simulink model "sparrow_albatros_spec_withgpio"  (R2021a)
settings: Solver=VariableStepDiscrete  StartTime=0.0  StopTime=100  RelTol=1e-3
undefined symbols (not defined in the file): pfb_coeff_gen_calc
libraries: xbsIndex_r4 x5582, casper_library_misc x33, casper_library_delays x28, xps_library x10, simulink x8, xbsReplacements_r4 x2
(part 55 of 80)

== system sparrow_albatros_spec_withgpio/fft_wideband_real/fft_biplex_real_4x/biplex_core/fft_stage_7/butterfly_direct/bus_norm0 ==
  din : Inport
  bussify : Subsystem  AncestorBlock=casper_library_flow_control/bus_create  mask(bus_create){inputNum=4}
      mask prompts: inputNum "Number of inputs:"
      mask init:
      | bus_create_init(gcb,...
      |     'inputNum', inputNum);
  conv{1..4} (4 alike) : xbsIndex_r4/Convert  gui_display_data_type=Fixed-point  arith_type="Signed  (2's comp)"  n_bits=27  bin_pt=18  float_type=Single  exp_bits=8  fraction_bits=24  quantization=Truncate  overflow=Wrap  en=off  latency=0  pipeline=on  dbl_ovrd=off  block_type=convert
  debus : Subsystem  AncestorBlock=casper_library_flow_control/bus_expand  mask(bus_expand){mode=divisions of arbitrary size, outputNum=2, outputWidth=[26 26 26 26], outputBinaryPt=[17 17 17 17], outputArithmeticType=[1 1 1 1], show_format=on, outputToWorkspace=off, variablePrefix=, outputToModelAsWell=on}
      mask prompts: outputNum "Number of outputs:"; outputWidth "Output width:"; outputBinaryPt "Output binary point position:"; outputArithmeticType "Output arithmetic type (ufix=0, fix=1, bool=2):"; show_format "Print format string?"; outputToWorkspace "Output to workspace?"; variablePrefix "Variable name prefix:"; outputToModelAsWell "Output to model as well?"
      mask help:
      | Expands a 'bus' made using a bus_create or Xilinx
      | concat block.
      | The input will be divided into the specified number
      | of outputs with the specified arithmetic types.
      | Divisions are made from most significant bit.
      mask init: same as sparrow_albatros_spec_withgpio/bus_expand
      settings: AttributesFormatString=4 outputs: f26.17,f26.17,f26.17,f26.17,
      mask TypeOptions mode: divisions of equal size | divisions of arbitrary size
      mask Callback mode: %bus_expand_callback();
      mask Callback outputWidth: %bus_expand_callback();
      mask Callback outputToWorkspace: %bus_expand_callback();
  dout : Outport
  wires:
  din/1 -> debus/1(bus_in)
  debus/1(msb_out4) -> conv1/1
  debus/2(out3) -> conv2/1
  debus/3(out2) -> conv3/1
  debus/4(lsb_out1) -> conv4/1
  conv1/1 -> bussify/1(in1)
  conv2/1 -> bussify/2(in2)
  conv3/1 -> bussify/3(in3)
  conv4/1 -> bussify/4(in4)
  bussify/1(bus_out) -> dout/1

== system sparrow_albatros_spec_withgpio/fft_wideband_real/fft_biplex_real_4x/biplex_core/fft_stage_7/butterfly_direct/bus_norm1 ==
  din : Inport
  bussify : Subsystem  AncestorBlock=casper_library_flow_control/bus_create  mask(bus_create){inputNum=4}
      mask prompts: inputNum "Number of inputs:"
      mask init:
      | bus_create_init(gcb,...
      |     'inputNum', inputNum);
  conv{1..4} (4 alike) : xbsIndex_r4/Convert  gui_display_data_type=Fixed-point  arith_type="Signed  (2's comp)"  n_bits=27  bin_pt=18  float_type=Single  exp_bits=8  fraction_bits=24  quantization=Truncate  overflow=Wrap  en=off  latency=0  pipeline=on  dbl_ovrd=off  block_type=convert
  debus : Subsystem  AncestorBlock=casper_library_flow_control/bus_expand  mask(bus_expand){mode=divisions of arbitrary size, outputNum=2, outputWidth=[26 26 26 26], outputBinaryPt=[18 18 18 18], outputArithmeticType=[1 1 1 1], show_format=on, outputToWorkspace=off, variablePrefix=, outputToModelAsWell=on}
      mask prompts: outputNum "Number of outputs:"; outputWidth "Output width:"; outputBinaryPt "Output binary point position:"; outputArithmeticType "Output arithmetic type (ufix=0, fix=1, bool=2):"; show_format "Print format string?"; outputToWorkspace "Output to workspace?"; variablePrefix "Variable name prefix:"; outputToModelAsWell "Output to model as well?"
      mask help:
      | Expands a 'bus' made using a bus_create or Xilinx
      | concat block.
      | The input will be divided into the specified number
      | of outputs with the specified arithmetic types.
      | Divisions are made from most significant bit.
      mask init: same as sparrow_albatros_spec_withgpio/bus_expand
      settings: AttributesFormatString=4 outputs: f26.18,f26.18,f26.18,f26.18,
      mask TypeOptions mode: divisions of equal size | divisions of arbitrary size
      mask Callback mode: %bus_expand_callback();
      mask Callback outputWidth: %bus_expand_callback();
      mask Callback outputToWorkspace: %bus_expand_callback();
  dout : Outport
  wires:
  din/1 -> debus/1(bus_in)
  debus/1(msb_out4) -> conv1/1
  debus/2(out3) -> conv2/1
  debus/3(out2) -> conv3/1
  debus/4(lsb_out1) -> conv4/1
  conv1/1 -> bussify/1(in1)
  conv2/1 -> bussify/2(in2)
  conv3/1 -> bussify/3(in3)
  conv4/1 -> bussify/4(in4)
  bussify/1(bus_out) -> dout/1

== system sparrow_albatros_spec_withgpio/fft_wideband_real/fft_biplex_real_4x/biplex_core/fft_stage_7/butterfly_direct/bus_relational ==
  a : Inport
  b : Inport  Port=2
  a_debus : Subsystem  AncestorBlock=casper_library_flow_control/bus_expand  mask(bus_expand){mode=divisions of arbitrary size, outputNum=2, outputWidth=[4], outputBinaryPt=[0], outputArithmeticType=[0], show_format=on, outputToWorkspace=off, variablePrefix=, outputToModelAsWell=on}
      mask prompts: outputNum "Number of outputs:"; outputWidth "Output width:"; outputBinaryPt "Output binary point position:"; outputArithmeticType "Output arithmetic type (ufix=0, fix=1, bool=2):"; show_format "Print format string?"; outputToWorkspace "Output to workspace?"; variablePrefix "Variable name prefix:"; outputToModelAsWell "Output to model as well?"
      mask help:
      | Expands a 'bus' made using a bus_create or Xilinx
      | concat block.
      | The input will be divided into the specified number
      | of outputs with the specified arithmetic types.
      | Divisions are made from most significant bit.
      mask init: same as sparrow_albatros_spec_withgpio/bus_expand
      settings: AttributesFormatString=1 outputs: uf4.0,
      mask TypeOptions mode: divisions of equal size | divisions of arbitrary size
      mask Callback mode: %bus_expand_callback();
      mask Callback outputWidth: %bus_expand_callback();
      mask Callback outputToWorkspace: %bus_expand_callback();
  b_debus : Subsystem  AncestorBlock=casper_library_flow_control/bus_expand  mask(bus_expand){mode=divisions of arbitrary size, outputNum=2, outputWidth=[4], outputBinaryPt=[0], outputArithmeticType=[0], show_format=on, outputToWorkspace=off, variablePrefix=, outputToModelAsWell=on}
      mask prompts: outputNum "Number of outputs:"; outputWidth "Output width:"; outputBinaryPt "Output binary point position:"; outputArithmeticType "Output arithmetic type (ufix=0, fix=1, bool=2):"; show_format "Print format string?"; outputToWorkspace "Output to workspace?"; variablePrefix "Variable name prefix:"; outputToModelAsWell "Output to model as well?"
      mask help:
      | Expands a 'bus' made using a bus_create or Xilinx
      | concat block.
      | The input will be divided into the specified number
      | of outputs with the specified arithmetic types.
      | Divisions are made from most significant bit.
      mask init: same as sparrow_albatros_spec_withgpio/bus_expand
      settings: AttributesFormatString=1 outputs: uf4.0,
      mask TypeOptions mode: divisions of equal size | divisions of arbitrary size
      mask Callback mode: %bus_expand_callback();
      mask Callback outputWidth: %bus_expand_callback();
      mask Callback outputToWorkspace: %bus_expand_callback();
  bussify : Subsystem  AncestorBlock=casper_library_flow_control/bus_create  mask(bus_create){inputNum=1}
      mask prompts: inputNum "Number of inputs:"
      mask init:
      | bus_create_init(gcb,...
      |     'inputNum', inputNum);
  relational1 : xbsIndex_r4/Relational  mode=a!=b  op_type=Bool  en=off  latency=1  dbl_ovrd=off  block_type=relational
  a!=b : Outport
  wires:
  a/1 -> a_debus/1(bus_in)
  b/1 -> b_debus/1(bus_in)
  a_debus/1(msb_lsb_out1) -> relational1/1
  b_debus/1(msb_lsb_out1) -> relational1/2
  relational1/1 -> bussify/1(in1)
  bussify/1(bus_out) -> a!=b/1

== system sparrow_albatros_spec_withgpio/fft_wideband_real/fft_biplex_real_4x/biplex_core/fft_stage_7/butterfly_direct/bus_scale ==
  din : Inport
  bussify : Subsystem  AncestorBlock=casper_library_flow_control/bus_create  mask(bus_create){inputNum=4}
      mask prompts: inputNum "Number of inputs:"
      mask init:
      | bus_create_init(gcb,...
      |     'inputNum', inputNum);
  debus : Subsystem  AncestorBlock=casper_library_flow_control/bus_expand  mask(bus_expand){mode=divisions of arbitrary size, outputNum=2, outputWidth=[26 26 26 26], outputBinaryPt=[17 17 17 17], outputArithmeticType=[1 1 1 1], show_format=on, outputToWorkspace=off, variablePrefix=, outputToModelAsWell=on}
      mask prompts: outputNum "Number of outputs:"; outputWidth "Output width:"; outputBinaryPt "Output binary point position:"; outputArithmeticType "Output arithmetic type (ufix=0, fix=1, bool=2):"; show_format "Print format string?"; outputToWorkspace "Output to workspace?"; variablePrefix "Variable name prefix:"; outputToModelAsWell "Output to model as well?"
      mask help:
      | Expands a 'bus' made using a bus_create or Xilinx
      | concat block.
      | The input will be divided into the specified number
      | of outputs with the specified arithmetic types.
      | Divisions are made from most significant bit.
      mask init: same as sparrow_albatros_spec_withgpio/bus_expand
      settings: AttributesFormatString=4 outputs: f26.17,f26.17,f26.17,f26.17,
      mask TypeOptions mode: divisions of equal size | divisions of arbitrary size
      mask Callback mode: %bus_expand_callback();
      mask Callback outputWidth: %bus_expand_callback();
      mask Callback outputToWorkspace: %bus_expand_callback();
  scale{1..4} (4 alike) : xbsIndex_r4/Scale  scale_factor=-1  dbl_ovrd=off  block_type=scale
  dout : Outport
  wires:
  din/1 -> debus/1(bus_in)
  debus/1(msb_out4) -> scale1/1
  debus/2(out3) -> scale2/1
  debus/3(out2) -> scale3/1
  debus/4(lsb_out1) -> scale4/1
  scale1/1 -> bussify/1(in1)
  scale2/1 -> bussify/2(in2)
  scale3/1 -> bussify/3(in3)
  scale4/1 -> bussify/4(in4)
  bussify/1(bus_out) -> dout/1

== system sparrow_albatros_spec_withgpio/fft_wideband_real/fft_biplex_real_4x/biplex_core/fft_stage_7/butterfly_direct/bus_sub ==
  a : Inport
  b : Inport  Port=2
  a_debus : Subsystem  AncestorBlock=casper_library_flow_control/bus_expand  mask(bus_expand){mode=divisions of arbitrary size, outputNum=2, outputWidth=[24  24], outputBinaryPt=[17  17], outputArithmeticType=[1  1], show_format=on, outputToWorkspace=off, variablePrefix=, outputToModelAsWell=on}
      mask prompts: outputNum "Number of outputs:"; outputWidth "Output width:"; outputBinaryPt "Output binary point position:"; outputArithmeticType "Output arithmetic type (ufix=0, fix=1, bool=2):"; show_format "Print format string?"; outputToWorkspace "Output to workspace?"; variablePrefix "Variable name prefix:"; outputToModelAsWell "Output to model as well?"
      mask help:
      | Expands a 'bus' made using a bus_create or Xilinx
      | concat block.
      | The input will be divided into the specified number
      | of outputs with the specified arithmetic types.
      | Divisions are made from most significant bit.
      mask init: same as sparrow_albatros_spec_withgpio/bus_expand
      settings: AttributesFormatString=2 outputs: f24.17,f24.17,
      mask TypeOptions mode: divisions of equal size | divisions of arbitrary size
      mask Callback mode: %bus_expand_callback();
      mask Callback outputWidth: %bus_expand_callback();
      mask Callback outputToWorkspace: %bus_expand_callback();
  addsub1 : xbsIndex_r4/AddSub  mode=Subtraction  use_carryin=off  use_carryout=off  en=off  latency=1  precision=User Defined  arith_type="Signed  (2's comp)"  n_bits=26  bin_pt=17  quantization=Truncate  overflow=Wrap  use_behavioral_HDL=on  hw_selection=Fabric  pipelined=on  dbl_ovrd=off  block_type=addsub
  addsub2 : xbsIndex_r4/AddSub  mode=Subtraction  use_carryin=off  use_carryout=off  en=off  latency=1  precision=User Defined  arith_type="Signed  (2's comp)"  n_bits=26  bin_pt=17  quantization=Truncate  overflow=Wrap  use_behavioral_HDL=on  hw_selection=Fabric  pipelined=on  dbl_ovrd=off  block_type=addsub
  b_debus : Subsystem  AncestorBlock=casper_library_flow_control/bus_expand  mask(bus_expand){mode=divisions of arbitrary size, outputNum=2, outputWidth=[25  25], outputBinaryPt=[17  17], outputArithmeticType=[1  1], show_format=on, outputToWorkspace=off, variablePrefix=, outputToModelAsWell=on}
      mask prompts: outputNum "Number of outputs:"; outputWidth "Output width:"; outputBinaryPt "Output binary point position:"; outputArithmeticType "Output arithmetic type (ufix=0, fix=1, bool=2):"; show_format "Print format string?"; outputToWorkspace "Output to workspace?"; variablePrefix "Variable name prefix:"; outputToModelAsWell "Output to model as well?"
      mask help:
      | Expands a 'bus' made using a bus_create or Xilinx
      | concat block.
      | The input will be divided into the specified number
      | of outputs with the specified arithmetic types.
      | Divisions are made from most significant bit.
      mask init: same as sparrow_albatros_spec_withgpio/bus_expand
      settings: AttributesFormatString=2 outputs: f25.17,f25.17,
      mask TypeOptions mode: divisions of equal size | divisions of arbitrary size
      mask Callback mode: %bus_expand_callback();
      mask Callback outputWidth: %bus_expand_callback();
      mask Callback outputToWorkspace: %bus_expand_callback();
  op_bussify : Subsystem  AncestorBlock=casper_library_flow_control/bus_create  mask(bus_create){inputNum=2}
      mask prompts: inputNum "Number of inputs:"
      mask init:
      | bus_create_init(gcb,...
      |     'inputNum', inputNum);
  dout : Outport
  wires:
  a/1 -> a_debus/1(bus_in)
  b/1 -> b_debus/1(bus_in)
  a_debus/1(msb_out2) -> addsub1/1
  b_debus/1(msb_out2) -> addsub1/2
  a_debus/2(lsb_out1) -> addsub2/1
  b_debus/2(lsb_out1) -> addsub2/2
  addsub1/1 -> op_bussify/1(in1)
  addsub2/1 -> op_bussify/2(in2)
  op_bussify/1(bus_out) -> dout/1

== system sparrow_albatros_spec_withgpio/fft_wideband_real/fft_biplex_real_4x/biplex_core/fft_stage_7/butterfly_direct/munge ==
  din : Inport
  join : Subsystem  AncestorBlock=casper_library_flow_control/bus_create  mask(bus_create){inputNum=2}
      mask prompts: inputNum "Number of inputs:"
      mask init:
      | bus_create_init(gcb,...
      |     'inputNum', inputNum);
  reinterpret : xbsIndex_r4/Reinterpret  force_arith_type=on  arith_type=Unsigned  force_bin_pt=on  bin_pt=0  block_type=reinterpret
  reinterpret_out : xbsIndex_r4/Reinterpret  force_arith_type=on  arith_type=Unsigned  force_bin_pt=on  bin_pt=0  block_type=reinterpret
  split : Subsystem  AncestorBlock=casper_library_flow_control/bus_expand  mask(bus_expand){mode=divisions of arbitrary size, outputNum=2, outputWidth=[2 2], outputBinaryPt=[0 0], outputArithmeticType=[0 0], show_format=off, outputToWorkspace=off, variablePrefix=out, outputToModelAsWell=on}
      mask prompts: outputNum "Number of outputs:"; outputWidth "Output width:"; outputBinaryPt "Output binary point position:"; outputArithmeticType "Output arithmetic type (ufix=0, fix=1, bool=2):"; show_format "Print format string?"; outputToWorkspace "Output to workspace?"; variablePrefix "Variable name prefix:"; outputToModelAsWell "Output to model as well?"
      mask help:
      | Expands a 'bus' made using a bus_create or Xilinx
      | concat block.
      | The input will be divided into the specified number
      | of outputs with the specified arithmetic types.
      | Divisions are made from most significant bit.
      mask init: same as sparrow_albatros_spec_withgpio/bus_expand
      settings: AttributesFormatString=2 outputs
      mask TypeOptions mode: divisions of equal size | divisions of arbitrary size
      mask Callback mode: %bus_expand_callback();
      mask Callback outputWidth: %bus_expand_callback();
      mask Callback outputToWorkspace: %bus_expand_callback();
  dout : Outport
  wires:
  reinterpret_out/1 -> dout/1
  din/1 -> reinterpret/1
  reinterpret/1 -> split/1(bus_in)
  join/1(bus_out) -> reinterpret_out/1
  split/1(msb_out2) -> join/1(in1)
  split/2(lsb_out1) -> join/2(in2)

== system sparrow_albatros_spec_withgpio/fft_wideband_real/fft_biplex_real_4x/biplex_core/fft_stage_7/butterfly_direct/mux ==
  sel : Inport
  d0 : Inport  Port=2
  d1 : Inport  Port=3
  d_bussify : Subsystem  AncestorBlock=casper_library_flow_control/bus_create  mask(bus_create){inputNum=4}
      mask prompts: inputNum "Number of inputs:"
      mask init:
      | bus_create_init(gcb,...
      |     'inputNum', inputNum);
  expand0 : Subsystem  AncestorBlock=casper_library_flow_control/bus_expand  mask(bus_expand){mode=divisions of arbitrary size, outputNum=2, outputWidth=[27 27 27 27], outputBinaryPt=[0  0  0  0], outputArithmeticType=[0  0  0  0], show_format=on, outputToWorkspace=off, variablePrefix=, outputToModelAsWell=on}
      mask prompts: outputNum "Number of outputs:"; outputWidth "Output width:"; outputBinaryPt "Output binary point position:"; outputArithmeticType "Output arithmetic type (ufix=0, fix=1, bool=2):"; show_format "Print format string?"; outputToWorkspace "Output to workspace?"; variablePrefix "Variable name prefix:"; outputToModelAsWell "Output to model as well?"
      mask help:
      | Expands a 'bus' made using a bus_create or Xilinx
      | concat block.
      | The input will be divided into the specified number
      | of outputs with the specified arithmetic types.
      | Divisions are made from most significant bit.
      mask init: same as sparrow_albatros_spec_withgpio/bus_expand
      settings: AttributesFormatString=4 outputs: uf27.0,uf27.0,uf27.0,uf27.0,
      mask TypeOptions mode: divisions of equal size | divisions of arbitrary size
      mask Callback mode: %bus_expand_callback();
      mask Callback outputWidth: %bus_expand_callback();
      mask Callback outputToWorkspace: %bus_expand_callback();
  expand1 : Subsystem  AncestorBlock=casper_library_flow_control/bus_expand  mask(bus_expand){mode=divisions of arbitrary size, outputNum=2, outputWidth=[27 27 27 27], outputBinaryPt=[0  0  0  0], outputArithmeticType=[0  0  0  0], show_format=on, outputToWorkspace=off, variablePrefix=, outputToModelAsWell=on}
      mask prompts: outputNum "Number of outputs:"; outputWidth "Output width:"; outputBinaryPt "Output binary point position:"; outputArithmeticType "Output arithmetic type (ufix=0, fix=1, bool=2):"; show_format "Print format string?"; outputToWorkspace "Output to workspace?"; variablePrefix "Variable name prefix:"; outputToModelAsWell "Output to model as well?"
      mask help:
      | Expands a 'bus' made using a bus_create or Xilinx
      | concat block.
      | The input will be divided into the specified number
      | of outputs with the specified arithmetic types.
      | Divisions are made from most significant bit.
      mask init: same as sparrow_albatros_spec_withgpio/bus_expand
      settings: AttributesFormatString=4 outputs: uf27.0,uf27.0,uf27.0,uf27.0,
      mask TypeOptions mode: divisions of equal size | divisions of arbitrary size
      mask Callback mode: %bus_expand_callback();
      mask Callback outputWidth: %bus_expand_callback();
      mask Callback outputToWorkspace: %bus_expand_callback();
  mux{0..3} (4 alike) : xbsIndex_r4/Mux  inputs=2  en=off  latency=1  precision=Full  arith_type=Unsigned  n_bits=16  bin_pt=14  quantization=Truncate  overflow=Wrap  dbl_ovrd=off  block_type=mux
  sel_expand : Subsystem  AncestorBlock=casper_library_flow_control/bus_expand  mask(bus_expand){mode=divisions of equal size, outputNum=4, outputWidth=1, outputBinaryPt=0, outputArithmeticType=0, show_format=on, outputToWorkspace=off, variablePrefix=, outputToModelAsWell=on}
      mask prompts: outputNum "Number of outputs:"; outputWidth "Output width:"; outputBinaryPt "Output binary point position:"; outputArithmeticType "Output arithmetic type (ufix=0, fix=1, bool=2):"; show_format "Print format string?"; outputToWorkspace "Output to workspace?"; variablePrefix "Variable name prefix:"; outputToModelAsWell "Output to model as well?"
      mask help:
      | Expands a 'bus' made using a bus_create or Xilinx
      | concat block.
      | The input will be divided into the specified number
      | of outputs with the specified arithmetic types.
      | Divisions are made from most significant bit.
      mask init: same as sparrow_albatros_spec_withgpio/bus_expand
      settings: AttributesFormatString=4 outputs: uf1.0,uf1.0,uf1.0,uf1.0,
      mask TypeOptions mode: divisions of equal size | divisions of arbitrary size
      mask Callback mode: %bus_expand_callback();
      mask Callback outputWidth: %bus_expand_callback();
      mask Callback outputToWorkspace: %bus_expand_callback();
  out : Outport
  wires:
  sel/1 -> sel_expand/1(bus_in)
  d0/1 -> expand0/1(bus_in)
  d1/1 -> expand1/1(bus_in)
  sel_expand/1(msb_out4) -> mux0/1
  expand0/1(msb_out4) -> mux0/2
  expand1/1(msb_out4) -> mux0/3
  sel_expand/2(out3) -> mux1/1
  expand0/2(out3) -> mux1/2
  expand1/2(out3) -> mux1/3
  sel_expand/3(out2) -> mux2/1
  expand0/3(out2) -> mux2/2
  expand1/3(out2) -> mux2/3
  sel_expand/4(lsb_out1) -> mux3/1
  expand0/4(lsb_out1) -> mux3/2
  expand1/4(lsb_out1) -> mux3/3
  mux0/1 -> d_bussify/1(in1)
  mux1/1 -> d_bussify/2(in2)
  mux2/1 -> d_bussify/3(in3)
  mux3/1 -> d_bussify/4(in4)
  d_bussify/1(bus_out) -> out/1

== system sparrow_albatros_spec_withgpio/fft_wideband_real/fft_biplex_real_4x/biplex_core/fft_stage_7/butterfly_direct/shift_replicate ==
  in : Inport
  bussify : Subsystem  AncestorBlock=casper_library_flow_control/bus_create  mask(bus_create){inputNum=4}
      mask prompts: inputNum "Number of inputs:"
      mask init:
      | bus_create_init(gcb,...
      |     'inputNum', inputNum);
  din0_{0..3} (4 alike) : xbsIndex_r4/Delay  rst=off  infoeditControl=Selection of Reset will increase slice count due to use of real FFs and instead of SRLs  en=off  latency=1  reg_retiming=off  dbl_ovrd=off  block_type=delay
  out : Outport
  wires:
  in/1 -> din0_0/1, din0_1/1, din0_2/1, din0_3/1
  din0_0/1 -> bussify/1(in1)
  din0_1/1 -> bussify/2(in2)
  din0_2/1 -> bussify/3(in3)
  din0_3/1 -> bussify/4(in4)
  bussify/1(bus_out) -> out/1

== system sparrow_albatros_spec_withgpio/fft_wideband_real/fft_biplex_real_4x/biplex_core/fft_stage_7/butterfly_direct/twiddle ==
  ai : Inport
  bi : Inport  Port=2
  sync_in : Inport  Port=3
  bus_convert : Subsystem  AncestorBlock=casper_library_bus/bus_convert  mask(bus_convert){n_bits_in=repmat(input_bit_width+coeff_bit_width+1, 1, n_inputs), bin_pt_in=(bin_pt_in+coeff_bit_width-1), cmplx=on, n_bits_out=input_bit_width+1, bin_pt_out=bin_pt_in, quantization=2, overflow=1, csp_latency=conv_latency, of=off, misc=on}
      mask prompts: n_bits_in "input bit widths"; bin_pt_in "input binary points"; cmplx "input complex"; n_bits_out "output bit widths"; bin_pt_out "output binary points"; quantization "quantization strategy (Truncate=0, Round  (unbiased: +/- Inf)=1, Round (unbiased: Even Values)=2)"; overflow "overflow strategy (Wrap=0, Saturate=1, Flag as error=2)"; csp_latency "latency"; of "overflow indication"; misc "misc support"
      mask help: Convert components of busses
      mask init: same as sparrow_albatros_spec_withgpio/tvg/bus_convert
  bus_create : Subsystem  AncestorBlock=casper_library_flow_control/bus_create  mask(bus_create){inputNum=3}
      mask prompts: inputNum "Number of inputs:"
      mask init:
      | bus_create_init(gcb,...
      |     'inputNum', inputNum);
  bus_expand : Subsystem  AncestorBlock=casper_library_flow_control/bus_expand  mask(bus_expand){mode=divisions of arbitrary size, outputNum=2, outputWidth=[n_inputs*input_bit_width*2, 1+(n_inputs*input_bit_width*2)], outputBinaryPt=[0 0], outputArithmeticType=[0 0], show_format=off, outputToWorkspace=off, variablePrefix=out, outputToModelAsWell=on}
      mask prompts: outputNum "Number of outputs:"; outputWidth "Output width:"; outputBinaryPt "Output binary point position:"; outputArithmeticType "Output arithmetic type (ufix=0, fix=1, bool=2):"; show_format "Print format string?"; outputToWorkspace "Output to workspace?"; variablePrefix "Variable name prefix:"; outputToModelAsWell "Output to model as well?"
      mask help:
      | Expands a 'bus' made using a bus_create or Xilinx
      | concat block.
      | The input will be divided into the specified number
      | of outputs with the specified arithmetic types.
      | Divisions are made from most significant bit.
      mask init: same as sparrow_albatros_spec_withgpio/bus_expand
      settings: AttributesFormatString=2 outputs
      mask TypeOptions mode: divisions of equal size | divisions of arbitrary size
      mask Callback mode: %bus_expand_callback();
      mask Callback outputWidth: %bus_expand_callback();
      mask Callback outputToWorkspace: %bus_expand_callback();
  bus_expand1 : Subsystem  AncestorBlock=casper_library_flow_control/bus_expand  mask(bus_expand){mode=divisions of arbitrary size, outputNum=2, outputWidth=[1 48], outputBinaryPt=[0 0], outputArithmeticType=[2 0], show_format=off, outputToWorkspace=off, variablePrefix=out, outputToModelAsWell=on}
      mask prompts: outputNum "Number of outputs:"; outputWidth "Output width:"; outputBinaryPt "Output binary point position:"; outputArithmeticType "Output arithmetic type (ufix=0, fix=1, bool=2):"; show_format "Print format string?"; outputToWorkspace "Output to workspace?"; variablePrefix "Variable name prefix:"; outputToModelAsWell "Output to model as well?"
      mask help:
      | Expands a 'bus' made using a bus_create or Xilinx
      | concat block.
      | The input will be divided into the specified number
      | of outputs with the specified arithmetic types.
      | Divisions are made from most significant bit.
      mask init: same as sparrow_albatros_spec_withgpio/bus_expand
      settings: AttributesFormatString=2 outputs
      mask TypeOptions mode: divisions of equal size | divisions of arbitrary size
      mask Callback mode: %bus_expand_callback();
      mask Callback outputWidth: %bus_expand_callback();
      mask Callback outputToWorkspace: %bus_expand_callback();
  bus_mult : Subsystem  AncestorBlock=casper_library_bus/bus_mult  mask(bus_mult){n_bits_a=coeff_bit_width, bin_pt_a=coeff_bit_width-1, type_a=1, cmplx_a=on, n_bits_b=24, bin_pt_b=bin_pt_in, type_b=1, cmplx_b=on, misc=on, floating_point=off, float_type=single, input_vec_a=1, input_vec_b=1, frac_width=24, exp_width=8, n_bits_out=input_bit_width+coeff_bit_width+1, bin_pt_out=(bin_pt_in+coeff_bit_width-1), type_out=1, quantization=0, overflow=0, mult_latency=mult_latency, add_latency=add_latency, conv_latency=0, max_fanout=max_fanout, fan_latency=0, multiplier_implementation=behavioral HDL, pipeline_cmult_en=off, pipeline_latency=0}
      mask prompts: n_bits_a "a input bit widths"; bin_pt_a "a input binary points"; type_a "a input type (Unsigned=0, Signed=1)"; cmplx_a "a input complex"; n_bits_b "b input bit widths"; bin_pt_b "b input binary points"; type_b "b input type (Unsigned=0, Signed=1)"; cmplx_b "b input complex"; misc "misc support"; floating_point "floating point"; float_type "float type"; input_vec_a "a input vector in bus"; input_vec_b "b input vector in bus"; frac_width "fraction width"; exp_width "exponent width"; n_bits_out "output bit widths"; bin_pt_out "output binary points"; type_out "output type (Unsigned=0, Signed=1)"; quantization "quantization strategy (Truncate=0, Round  (unbiased: +/- Inf)=1, , Round  (unbiased: Even Values)=2)"; overflow "overflow strategy (Wrap=0, Saturate=1, Flag as error=2)"; mult_latency "multiplier latency"; add_latency "adder latency"; conv_latency "convert latency"; max_fanout "limit fanout to ?"; fan_latency "fanout register latency"; multiplier_implementation "multiplier implementation"; pipeline_cmult_en "pipeline complex mult"; pipeline_latency "pipeline latency"
      mask help: Multiply components of two busses
      mask init: same as sparrow_albatros_spec_withgpio/fft_wideband_real/fft_direct/butterfly0_0/twiddle/bus_mult
      mask Callback floating_point:
      | onoff = get_param(gcb, 'floating_point');
      | if strcmp(onoff,'on')
      |     enable_fixpt = 'off';
      |     set_param_state(gcb, 'float_type', 'on')
      | 
      |     set_param_state(gcb, 'input_vec_a', 'on')
      |     set_param_state(gcb, 'input_vec_b', 'on')
      | 
      |     f_type = get_param(gcb, 'float_type');
      |     if strcmp(f_type,'custom')
      |         set_param_state(gcb, 'exp_width', 'on')
      |         set_param_state(gcb, 'frac_width', 'on')
      |     else
      |         set_param_state(gcb, 'exp_width', 'off')
      |         set_param_state(gcb, 'frac_width', 'off')
      |     end
      | 
      | else
      |     enable_fixpt = 'on';
      |     set_param_state(gcb, 'float_type', 'off')
      |     set_param_state(gcb, 'exp_width', 'off')
      |     set_param_state(gcb, 'frac_width', 'off')
      |     set_param_state(gcb, 'input_vec_a', 'off')
      |     set_param_state(gcb, 'input_vec_b', 'off')
      | end
      | 
      | set_param_state(gcb, 'n_bits_a', enable_fixpt)
      | set_param_state(gcb, 'bin_pt_a', enable_fixpt)
      | set_param_state(gcb, 'type_a', enable_fixpt)
      | set_param_state(gcb, 'n_bits_b', enable_fixpt)
      | set_param_state(gcb, 'bin_pt_b', enable_fixpt)
      | set_param_state(gcb, 'type_b', enable_fixpt)
      | 
      | set_param_state(gcb, 'n_bits_out', enable_fixpt)
      | set_param_state(gcb, 'bin_pt_out', enable_fixpt)
      | set_param_state(gcb, 'type_out', enable_fixpt)
      | set_param_state(gcb, 'quantization', enable_fixpt)
      | set_param_state(gcb, 'overflow', enable_fixpt)
      mask TypeOptions float_type: single | custom
      mask Callback float_type:
      | f_type = get_param(gcb, 'float_type');
      | if strcmp(f_type,'custom')
      |     set_param_state(gcb, 'exp_width', 'on')
      |     set_param_state(gcb, 'frac_width', 'on')
      | else
      |     set_param_state(gcb, 'exp_width', 'off')
      |     set_param_state(gcb, 'frac_width', 'off')
      | end
      mask TypeOptions multiplier_implementation: behavioral HDL | standard core | embedded multiplier core
      mask Callback pipeline_cmult_en:
      | pipeline_en = get_param(gcb, 'pipeline_cmult_en');
      | if strcmp(pipeline_en,'on')
      | 
      |     set_param_state(gcb, 'pipeline_latency', 'on')
      | else
      |     set_param_state(gcb, 'pipeline_latency', 'off')
      | end
  coeff_gen : Subsystem  AncestorBlock=casper_library_ffts_twiddle_coeff_gen/coeff_gen  mask(coeff_gen){FFTSize=FFTSize, Coeffs=[0 1 2 3 4 5 6 7 8 9 10 11 12 13 14 15 16 17 18 19 20 21 22 23 24 25 26 27 28 29 30 31 32 33 34 35 36 37 38 39 40 41 42 43 44 45 46 47 48 49 50 51 52 53 54 55 56 57 58 59 60 61 62 63], coeff_bit_width=coeff_bit_width, StepPeriod=StepPeriod, async=off, misc=on, floating_point=off, float_type=single, exp_width=8, frac_width=24, bram_latency=bram_latency, mult_latency=mult_latency, add_latency=add_latency, conv_latency=conv_latency, coeffs_bit_limit=coeffs_bit_limit, coeff_sharing=on, coeff_decimation=on, coeff_generation=off, cal_bits=cal_bits, n_bits_rotation=n_bits_rotation, quantization=Round  (unbiased: Even Values)}
      mask prompts: FFTSize "fft size (2^?)"; Coeffs "Coefficients"; coeff_bit_width "Coefficient Bit Width:"; StepPeriod "Step Period: (2^?)"; async "asynchronous operation"; misc "misc port"; floating_point "floating point"; exp_width "exponential width"; frac_width "fractional width"; bram_latency "BRAM latency"; mult_latency "Multiplier latency"; add_latency "Adder latency"; conv_latency "Convert latency"; coeffs_bit_limit "Number bits above which to store stage's coefficients in BRAM (2^? bits)"; coeff_sharing "BRAM sharing in coeff storage"; coeff_decimation "Store a fraction of coeff factors where useful"; coeff_generation "Generate coeffs with multipliers where useful"; cal_bits "Number calibration locations when generating coeffs (2^?)"; n_bits_rotation "Rotation vector resolution"; quantization "Quantization strategy"
      mask help:
      | Generates a sequence of complex coefficients for use in generating twiddle
      | factors for FFTs.
      mask init: same as sparrow_albatros_spec_withgpio/fft_wideband_real/fft_direct/butterfly0_0/twiddle/coeff_gen
      settings: AttributesFormatString=64 @ (18,17)
      mask Callback floating_point:
      | onoff = get_param(gcb, 'floating_point');
      | if strcmp(onoff,'on')
      |     enable_fixpt = 'off';
      |     set_param_state(gcb, 'float_type', 'on')
      | 
      |     f_type = get_param(gcb, 'float_type');
      |     if strcmp(f_type,'custom')
      |         set_param_state(gcb, 'exp_width', 'on')
      |         set_param_state(gcb, 'frac_width', 'on')
      |     else
      |         set_param_state(gcb, 'exp_width', 'off')
      |         set_param_state(gcb, 'frac_width', 'off')
      |     end
      | 
      | 
      | else
      |     enable_fixpt = 'on';
      |     set_param_state(gcb, 'float_type', 'off')
      |     set_param_state(gcb, 'exp_width', 'off')
      |     set_param_state(gcb, 'frac_width', 'off')
      | end
      mask TypeOptions float_type: single | custom
      mask Callback float_type:
      | f_type = get_param(gcb, 'float_type');
      | if strcmp(f_type,'custom')
      |     set_param_state(gcb, 'exp_width', 'on')
      |     set_param_state(gcb, 'frac_width', 'on')
      | else
      |     set_param_state(gcb, 'exp_width', 'off')
      |     set_param_state(gcb, 'frac_width', 'off')
      | end
      mask TypeOptions quantization: Truncate | Round  (unbiased: +/- Inf) | Round  (unbiased: Even Values)
      mask DialogControl ParameterTabVar0 Prompt: basic
      mask DialogControl ParameterTabVar01 Prompt: latency
      mask DialogControl ParameterTabVar012 Prompt: implementation
  ao : Outport
  bwo : Outport  Port=2
  sync_out : Outport  Port=3
  wires:
  bi/1 -> bus_create/1(in1)
  sync_in/1 -> bus_create/2(in2), coeff_gen/1(rst)
  ai/1 -> bus_create/3(in3)
  bus_create/1(bus_out) -> coeff_gen/2(misci)
  coeff_gen/2(misco) -> bus_expand/1(bus_in)
  coeff_gen/1(w) -> bus_mult/1(a)
  bus_expand/2(lsb_out1) -> bus_mult/3(misci)
  bus_expand/1(msb_out2) -> bus_mult/2(b)
  bus_mult/1(a*b) -> bus_convert/1(din)
  bus_mult/2(misco) -> bus_convert/2(misci)
  bus_convert/1(dout) -> bwo/1
  bus_convert/2(misco) -> bus_expand1/1(bus_in)
  bus_expand1/1(msb_out2) -> sync_out/1
  bus_expand1/2(lsb_out1) -> ao/1

== system sparrow_albatros_spec_withgpio/fft_wideband_real/fft_biplex_real_4x/biplex_core/fft_stage_7/delay0/din_expand ==
  bus_in : Inport
  reinterpret1 : xbsIndex_r4/Reinterpret  force_arith_type=on  arith_type=Unsigned  force_bin_pt=on  bin_pt=0  block_type=reinterpret
  slice1 : xbsIndex_r4/Slice  nbits=48  boolean_output=off  mode=Upper Bit Location + Width  bit1=0  base1=MSB of Input  bit0=0  base0=LSB of Input  dbl_ovrd=off  block_type=slice
  msb_lsb_out1 : Outport
  wires:
  bus_in/1 -> slice1/1
  slice1/1 -> reinterpret1/1
  reinterpret1/1 -> msb_lsb_out1/1

== system sparrow_albatros_spec_withgpio/fft_wideband_real/fft_biplex_real_4x/biplex_core/fft_stage_7/delay0/dout_compress ==
  in1 : Inport
  reinterpret1 : xbsIndex_r4/Reinterpret  force_arith_type=on  arith_type=Unsigned  force_bin_pt=on  bin_pt=0  block_type=reinterpret
      settings: infoedit="Changes signal type without altering the binary representation.   You can changed the signal between signed and unsigned, and relocate the binary point.<br><br>Hardware notes: In hardware this block costs nothing.<br><br>Example:  Suppose the input is 6 bits wide, signed, with 2 fractional bits, and the output is forced to unsigned with 0 fractional bits.  Then an input of -2.0 (1110.00 in binary 2's complement) becomes an output of 56 (111000 in binary)."
  bus_out : Outport  VectorParamsAs1DForOutWhenUnconnected=off
  wires:
  in1/1 -> reinterpret1/1
  reinterpret1/1 -> bus_out/1

== system sparrow_albatros_spec_withgpio/fft_wideband_real/fft_biplex_real_4x/biplex_core/fft_stage_7/delay1/din_expand ==
  bus_in : Inport
  reinterpret1 : xbsIndex_r4/Reinterpret  force_arith_type=on  arith_type=Unsigned  force_bin_pt=on  bin_pt=0  block_type=reinterpret
  slice1 : xbsIndex_r4/Slice  nbits=48  boolean_output=off  mode=Upper Bit Location + Width  bit1=0  base1=MSB of Input  bit0=0  base0=LSB of Input  dbl_ovrd=off  block_type=slice
  msb_lsb_out1 : Outport
  wires:
  bus_in/1 -> slice1/1
  slice1/1 -> reinterpret1/1
  reinterpret1/1 -> msb_lsb_out1/1

== system sparrow_albatros_spec_withgpio/fft_wideband_real/fft_biplex_real_4x/biplex_core/fft_stage_7/delay1/dout_compress ==
  in1 : Inport
  reinterpret1 : xbsIndex_r4/Reinterpret  force_arith_type=on  arith_type=Unsigned  force_bin_pt=on  bin_pt=0  block_type=reinterpret
      settings: infoedit="Changes signal type without altering the binary representation.   You can changed the signal between signed and unsigned, and relocate the binary point.<br><br>Hardware notes: In hardware this block costs nothing.<br><br>Example:  Suppose the input is 6 bits wide, signed, with 2 fractional bits, and the output is forced to unsigned with 0 fractional bits.  Then an input of -2.0 (1110.00 in binary 2's complement) becomes an output of 56 (111000 in binary)."
  bus_out : Outport  VectorParamsAs1DForOutWhenUnconnected=off
  wires:
  in1/1 -> reinterpret1/1
  reinterpret1/1 -> bus_out/1

== system sparrow_albatros_spec_withgpio/fft_wideband_real/fft_biplex_real_4x/biplex_core/fft_stage_8/butterfly_direct/bus_add ==
  a : Inport
  b : Inport  Port=2
  a_debus : Subsystem  AncestorBlock=casper_library_flow_control/bus_expand  mask(bus_expand){mode=divisions of arbitrary size, outputNum=2, outputWidth=[24  24], outputBinaryPt=[17  17], outputArithmeticType=[1  1], show_format=on, outputToWorkspace=off, variablePrefix=, outputToModelAsWell=on}
      mask prompts: outputNum "Number of outputs:"; outputWidth "Output width:"; outputBinaryPt "Output binary point position:"; outputArithmeticType "Output arithmetic type (ufix=0, fix=1, bool=2):"; show_format "Print format string?"; outputToWorkspace "Output to workspace?"; variablePrefix "Variable name prefix:"; outputToModelAsWell "Output to model as well?"
      mask help:
      | Expands a 'bus' made using a bus_create or Xilinx
      | concat block.
      | The input will be divided into the specified number
      | of outputs with the specified arithmetic types.
      | Divisions are made from most significant bit.
      mask init: same as sparrow_albatros_spec_withgpio/bus_expand
      settings: AttributesFormatString=2 outputs: f24.17,f24.17,
      mask TypeOptions mode: divisions of equal size | divisions of arbitrary size
      mask Callback mode: %bus_expand_callback();
      mask Callback outputWidth: %bus_expand_callback();
      mask Callback outputToWorkspace: %bus_expand_callback();
  addsub1 : xbsIndex_r4/AddSub  mode=Addition  use_carryin=off  use_carryout=off  en=off  latency=1  precision=User Defined  arith_type="Signed  (2's comp)"  n_bits=26  bin_pt=17  quantization=Truncate  overflow=Wrap  use_behavioral_HDL=on  hw_selection=Fabric  pipelined=on  dbl_ovrd=off  block_type=addsub
  addsub2 : xbsIndex_r4/AddSub  mode=Addition  use_carryin=off  use_carryout=off  en=off  latency=1  precision=User Defined  arith_type="Signed  (2's comp)"  n_bits=26  bin_pt=17  quantization=Truncate  overflow=Wrap  use_behavioral_HDL=on  hw_selection=Fabric  pipelined=on  dbl_ovrd=off  block_type=addsub
  b_debus : Subsystem  AncestorBlock=casper_library_flow_control/bus_expand  mask(bus_expand){mode=divisions of arbitrary size, outputNum=2, outputWidth=[25  25], outputBinaryPt=[17  17], outputArithmeticType=[1  1], show_format=on, outputToWorkspace=off, variablePrefix=, outputToModelAsWell=on}
      mask prompts: outputNum "Number of outputs:"; outputWidth "Output width:"; outputBinaryPt "Output binary point position:"; outputArithmeticType "Output arithmetic type (ufix=0, fix=1, bool=2):"; show_format "Print format string?"; outputToWorkspace "Output to workspace?"; variablePrefix "Variable name prefix:"; outputToModelAsWell "Output to model as well?"
      mask help:
      | Expands a 'bus' made using a bus_create or Xilinx
      | concat block.
      | The input will be divided into the specified number
      | of outputs with the specified arithmetic types.
      | Divisions are made from most significant bit.
      mask init: same as sparrow_albatros_spec_withgpio/bus_expand
      settings: AttributesFormatString=2 outputs: f25.17,f25.17,
      mask TypeOptions mode: divisions of equal size | divisions of arbitrary size
      mask Callback mode: %bus_expand_callback();
      mask Callback outputWidth: %bus_expand_callback();
      mask Callback outputToWorkspace: %bus_expand_callback();
  op_bussify : Subsystem  AncestorBlock=casper_library_flow_control/bus_create  mask(bus_create){inputNum=2}
      mask prompts: inputNum "Number of inputs:"
      mask init:
      | bus_create_init(gcb,...
      |     'inputNum', inputNum);
  dout : Outport
  wires:
  a/1 -> a_debus/1(bus_in)
  b/1 -> b_debus/1(bus_in)
  a_debus/1(msb_out2) -> addsub1/1
  b_debus/1(msb_out2) -> addsub1/2
  a_debus/2(lsb_out1) -> addsub2/1
  b_debus/2(lsb_out1) -> addsub2/2
  addsub1/1 -> op_bussify/1(in1)
  addsub2/1 -> op_bussify/2(in2)
  op_bussify/1(bus_out) -> dout/1

== system sparrow_albatros_spec_withgpio/fft_wideband_real/fft_biplex_real_4x/biplex_core/fft_stage_8/butterfly_direct/bus_convert ==
  din : Inport
  bussify : Subsystem  AncestorBlock=casper_library_flow_control/bus_create  mask(bus_create){inputNum=4}
      mask prompts: inputNum "Number of inputs:"
      mask init:
      | bus_create_init(gcb,...
      |     'inputNum', inputNum);
  conv1 : Subsystem  AncestorBlock=casper_library_misc/convert_of  mask(convert_of){bit_width_i=27, binary_point_i=18, bit_width_o=24, binary_point_o=17, csp_latency=1, overflow=Saturate, quantization=Round  (unbiased: even values)}
      mask prompts: bit_width_i "Bit Width In"; binary_point_i "Binary Point In"; bit_width_o "Bit Width Out"; binary_point_o "Binary Point Out"; csp_latency "Latency"; overflow "Overflow Behaviour"; quantization "Quantization Behaviour"
      mask help:
      | Converts from one 2's complement bit-width
      | and/or binary point position to another.
      | Includes underflow/overflow indicator.
      mask init: same as sparrow_albatros_spec_withgpio/fft_wideband_real/fft_direct/butterfly0_0/bus_convert/conv1
      settings: AttributesFormatString=[27,18]->[24,17]
      mask TypeOptions overflow: Wrap | Saturate | Error
      mask TypeOptions quantization: Truncate | Round  (unbiased: +/- Inf) | Round  (unbiased: even values)
  conv2 : Subsystem  AncestorBlock=casper_library_misc/convert_of  mask(convert_of){bit_width_i=27, binary_point_i=18, bit_width_o=24, binary_point_o=17, csp_latency=1, overflow=Saturate, quantization=Round  (unbiased: even values)}
      mask prompts: bit_width_i "Bit Width In"; binary_point_i "Binary Point In"; bit_width_o "Bit Width Out"; binary_point_o "Binary Point Out"; csp_latency "Latency"; overflow "Overflow Behaviour"; quantization "Quantization Behaviour"
      mask help:
      | Converts from one 2's complement bit-width
      | and/or binary point position to another.
      | Includes underflow/overflow indicator.
      mask init: same as sparrow_albatros_spec_withgpio/fft_wideband_real/fft_direct/butterfly0_0/bus_convert/conv1
      settings: AttributesFormatString=[27,18]->[24,17]
      mask TypeOptions overflow: Wrap | Saturate | Error
      mask TypeOptions quantization: Truncate | Round  (unbiased: +/- Inf) | Round  (unbiased: even values)
  conv3 : Subsystem  AncestorBlock=casper_library_misc/convert_of  mask(convert_of){bit_width_i=27, binary_point_i=18, bit_width_o=24, binary_point_o=17, csp_latency=1, overflow=Saturate, quantization=Round  (unbiased: even values)}
      mask prompts: bit_width_i "Bit Width In"; binary_point_i "Binary Point In"; bit_width_o "Bit Width Out"; binary_point_o "Binary Point Out"; csp_latency "Latency"; overflow "Overflow Behaviour"; quantization "Quantization Behaviour"
      mask help:
      | Converts from one 2's complement bit-width
      | and/or binary point position to another.
      | Includes underflow/overflow indicator.
      mask init: same as sparrow_albatros_spec_withgpio/fft_wideband_real/fft_direct/butterfly0_0/bus_convert/conv1
      settings: AttributesFormatString=[27,18]->[24,17]
      mask TypeOptions overflow: Wrap | Saturate | Error
      mask TypeOptions quantization: Truncate | Round  (unbiased: +/- Inf) | Round  (unbiased: even values)
  conv4 : Subsystem  AncestorBlock=casper_library_misc/convert_of  mask(convert_of){bit_width_i=27, binary_point_i=18, bit_width_o=24, binary_point_o=17, csp_latency=1, overflow=Saturate, quantization=Round  (unbiased: even values)}
      mask prompts: bit_width_i "Bit Width In"; binary_point_i "Binary Point In"; bit_width_o "Bit Width Out"; binary_point_o "Binary Point Out"; csp_latency "Latency"; overflow "Overflow Behaviour"; quantization "Quantization Behaviour"
      mask help:
      | Converts from one 2's complement bit-width
      | and/or binary point position to another.
      | Includes underflow/overflow indicator.
      mask init: same as sparrow_albatros_spec_withgpio/fft_wideband_real/fft_direct/butterfly0_0/bus_convert/conv1
      settings: AttributesFormatString=[27,18]->[24,17]
      mask TypeOptions overflow: Wrap | Saturate | Error
      mask TypeOptions quantization: Truncate | Round  (unbiased: +/- Inf) | Round  (unbiased: even values)
  debus : Subsystem  AncestorBlock=casper_library_flow_control/bus_expand  mask(bus_expand){mode=divisions of arbitrary size, outputNum=2, outputWidth=[27 27 27 27], outputBinaryPt=[18 18 18 18], outputArithmeticType=[1 1 1 1], show_format=on, outputToWorkspace=off, variablePrefix=, outputToModelAsWell=on}
      mask prompts: outputNum "Number of outputs:"; outputWidth "Output width:"; outputBinaryPt "Output binary point position:"; outputArithmeticType "Output arithmetic type (ufix=0, fix=1, bool=2):"; show_format "Print format string?"; outputToWorkspace "Output to workspace?"; variablePrefix "Variable name prefix:"; outputToModelAsWell "Output to model as well?"
      mask help:
      | Expands a 'bus' made using a bus_create or Xilinx
      | concat block.
      | The input will be divided into the specified number
      | of outputs with the specified arithmetic types.
      | Divisions are made from most significant bit.
      mask init: same as sparrow_albatros_spec_withgpio/bus_expand
      settings: AttributesFormatString=4 outputs: f27.18,f27.18,f27.18,f27.18,
      mask TypeOptions mode: divisions of equal size | divisions of arbitrary size
      mask Callback mode: %bus_expand_callback();
      mask Callback outputWidth: %bus_expand_callback();
      mask Callback outputToWorkspace: %bus_expand_callback();
  of_bussify : Subsystem  AncestorBlock=casper_library_flow_control/bus_create  mask(bus_create){inputNum=4}
      mask prompts: inputNum "Number of inputs:"
      mask init:
      | bus_create_init(gcb,...
      |     'inputNum', inputNum);
  dout : Outport
  overflow : Outport  Port=2
  wires:
  din/1 -> debus/1(bus_in)
  debus/1(msb_out4) -> conv1/1(din)
  debus/2(out3) -> conv2/1(din)
  debus/3(out2) -> conv3/1(din)
  debus/4(lsb_out1) -> conv4/1(din)
  conv1/1(dout) -> bussify/1(in1)
  conv2/1(dout) -> bussify/2(in2)
  conv3/1(dout) -> bussify/3(in3)
  conv4/1(dout) -> bussify/4(in4)
  conv1/2(of) -> of_bussify/1(in1)
  conv2/2(of) -> of_bussify/2(in2)
  conv3/2(of) -> of_bussify/3(in3)
  conv4/2(of) -> of_bussify/4(in4)
  bussify/1(bus_out) -> dout/1
  of_bussify/1(bus_out) -> overflow/1

== system sparrow_albatros_spec_withgpio/fft_wideband_real/fft_biplex_real_4x/biplex_core/fft_stage_8/butterfly_direct/bus_expand ==
  bus_in : Inport
  reinterpret1 : xbsIndex_r4/Reinterpret  force_arith_type=on  arith_type=Unsigned  force_bin_pt=on  bin_pt=0  block_type=reinterpret
  reinterpret2 : xbsIndex_r4/Reinterpret  force_arith_type=on  arith_type=Unsigned  force_bin_pt=on  bin_pt=0  block_type=reinterpret
  slice1 : xbsIndex_r4/Slice  nbits=48  boolean_output=off  mode=Upper Bit Location + Width  bit1=-48  base1=MSB of Input  bit0=0  base0=LSB of Input  dbl_ovrd=off  block_type=slice
  slice2 : xbsIndex_r4/Slice  nbits=48  boolean_output=off  mode=Upper Bit Location + Width  bit1=0  base1=MSB of Input  bit0=0  base0=LSB of Input  dbl_ovrd=off  block_type=slice
  msb_out2 : Outport  VectorParamsAs1DForOutWhenUnconnected=off
  lsb_out1 : Outport  Port=2  VectorParamsAs1DForOutWhenUnconnected=off
  wires:
  bus_in/1 -> slice2/1, slice1/1
  slice2/1 -> reinterpret2/1
  reinterpret2/1 -> msb_out2/1
  slice1/1 -> reinterpret1/1
  reinterpret1/1 -> lsb_out1/1
